simulink model "simulink_LenkmomentB"  (Simulink 6.5)
settings: Solver=ode5  StartTime=0.0  StopTime=15  FixedStep=0.001  RelTol=1e-3
PreLoadFcn:
  | global d
  | global p
undefined symbols (not defined in the file or in its folder): d, p, x
settings Model: Creator=tftbe1  LastModifiedBy=localadmin
settings OptimizationCC: InitFltsAndDblsToZero=off
settings DebuggingCC: SignalResolutionControl=UseLocalSettings  StrictBusMsg=ErrorLevel1
settings GRTTargetCC: TargetFcnLib=ansi_tfl_table_tmw.mat

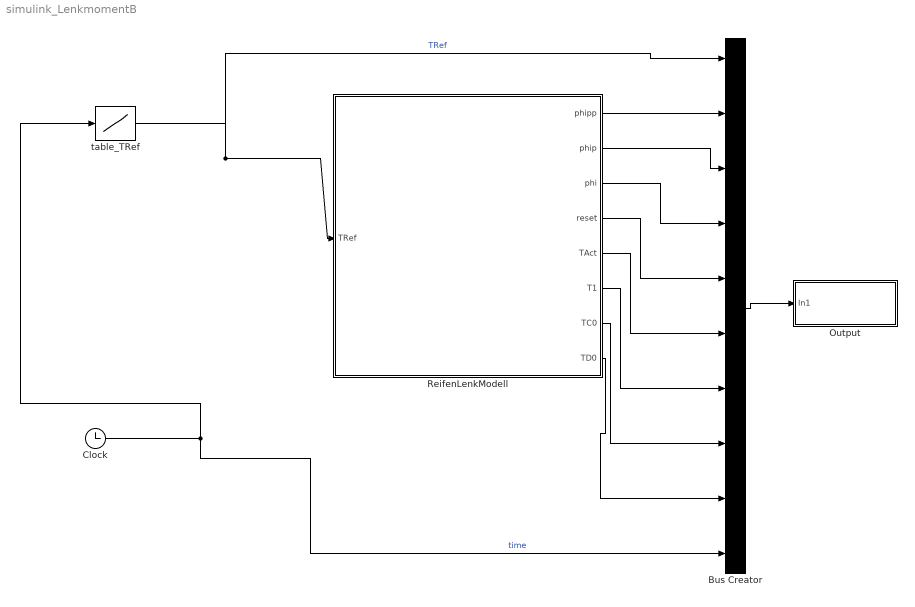
== system simulink_LenkmomentB ==
  Bus Creator : BusCreator  Inputs=10
  Clock : Clock
      settings: Decimation=10
  Output : Subsystem
  ReifenLenkModell : Subsystem
  table_TRef : Lookup  InputValues=d.time  OutputValues=d.IPAS_Soll_Lenkmoment  LookUpMeth=Interpolation-Extrapolation  OutDataType=sfix(16)  OutScaling=2^0  SampleTime=-1  LUTDesignTableMode=Redesign Table  LUTDesignDataSource=Block Dialog  LUTDesignFunctionName=sqrt(x)  LUTDesignUseExistingBP=on  LUTDesignRelError=0.01  LUTDesignAbsError=1e-6  SaturateOnIntegerOverflow=off  RndMeth=Floor
      settings: LockScale=off
  wires:
  Bus Creator/1 -> Output/1(In1)
  ReifenLenkModell/1(phipp) -> Bus Creator/2
  ReifenLenkModell/2(phip) -> Bus Creator/3
  ReifenLenkModell/3(phi) -> Bus Creator/4
  Clock/1 -> table_TRef/1, Bus Creator/10  "time"
  table_TRef/1 -> ReifenLenkModell/1(TRef), Bus Creator/1  "TRef"
  ReifenLenkModell/4(reset) -> Bus Creator/5
  ReifenLenkModell/5(TAct) -> Bus Creator/6
  ReifenLenkModell/6(T1) -> Bus Creator/7
  ReifenLenkModell/7(TC0) -> Bus Creator/8
  ReifenLenkModell/8(TD0) -> Bus Creator/9

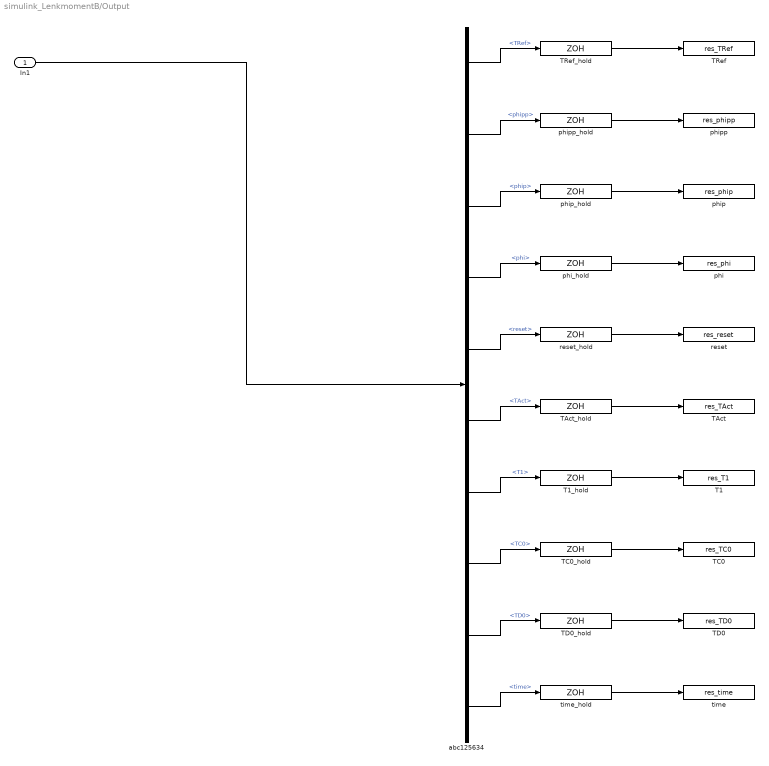
== system simulink_LenkmomentB/Output ==
  In1 : Inport
  T1 : ToWorkspace  VariableName=res_T1  SampleTime=-1  SaveFormat=Array
  T1_hold : ZeroOrderHold  SampleTime=0.01
  TAct : ToWorkspace  VariableName=res_TAct  SampleTime=-1  SaveFormat=Array
  TAct_hold : ZeroOrderHold  SampleTime=0.01
  TC0 : ToWorkspace  VariableName=res_TC0  SampleTime=-1  SaveFormat=Array
  TC0_hold : ZeroOrderHold  SampleTime=0.01
  TD0 : ToWorkspace  VariableName=res_TD0  SampleTime=-1  SaveFormat=Array
  TD0_hold : ZeroOrderHold  SampleTime=0.01
  TRef : ToWorkspace  VariableName=res_TRef  SampleTime=-1  SaveFormat=Array
  TRef_hold : ZeroOrderHold  SampleTime=0.01
  abc125634 : BusSelector  OutputSignals=TRef,phipp,phip,phi,reset,TAct,T1,TC0,TD0,time
  phi : ToWorkspace  VariableName=res_phi  SampleTime=-1  SaveFormat=Array
  phi_hold : ZeroOrderHold  SampleTime=0.01
  phip : ToWorkspace  VariableName=res_phip  SampleTime=-1  SaveFormat=Array
  phip_hold : ZeroOrderHold  SampleTime=0.01
  phipp : ToWorkspace  VariableName=res_phipp  SampleTime=-1  SaveFormat=Array
  phipp_hold : ZeroOrderHold  SampleTime=0.01
  reset : ToWorkspace  VariableName=res_reset  SampleTime=-1  SaveFormat=Array
  reset_hold : ZeroOrderHold  SampleTime=0.01
  time : ToWorkspace  VariableName=res_time  SampleTime=-1  SaveFormat=Array
  time_hold : ZeroOrderHold  SampleTime=0.01
  wires:
  In1/1 -> abc125634/1
  abc125634/1 -> TRef_hold/1  "<TRef>"
  TRef_hold/1 -> TRef/1
  abc125634/2 -> phipp_hold/1  "<phipp>"
  phipp_hold/1 -> phipp/1
  abc125634/3 -> phip_hold/1  "<phip>"
  phip_hold/1 -> phip/1
  abc125634/4 -> phi_hold/1  "<phi>"
  phi_hold/1 -> phi/1
  abc125634/5 -> reset_hold/1  "<reset>"
  reset_hold/1 -> reset/1
  abc125634/6 -> TAct_hold/1  "<TAct>"
  TAct_hold/1 -> TAct/1
  abc125634/7 -> T1_hold/1  "<T1>"
  T1_hold/1 -> T1/1
  abc125634/8 -> TC0_hold/1  "<TC0>"
  TC0_hold/1 -> TC0/1
  abc125634/9 -> TD0_hold/1  "<TD0>"
  TD0_hold/1 -> TD0/1
  abc125634/10 -> time_hold/1  "<time>"
  time_hold/1 -> time/1

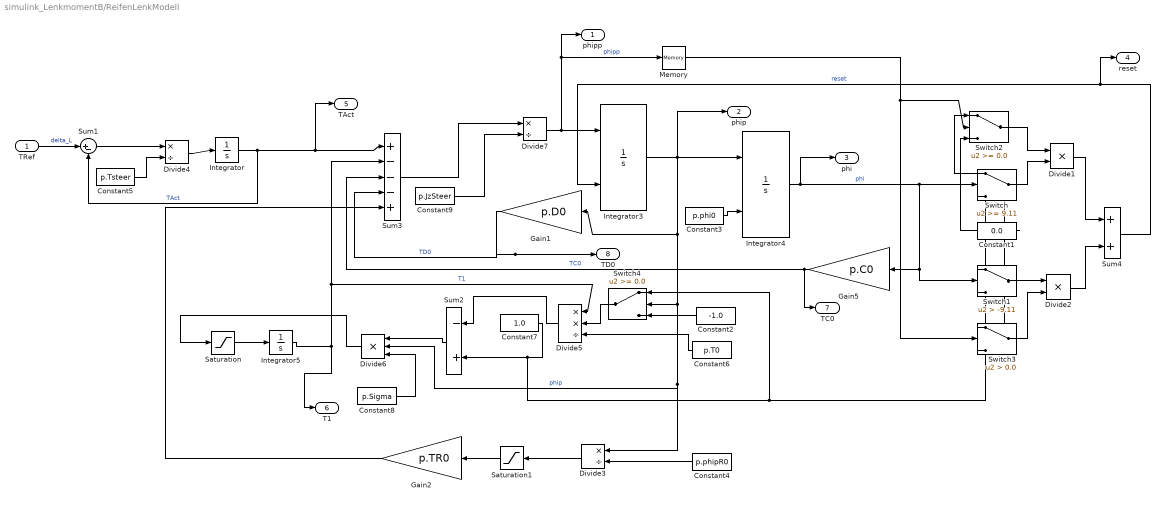
== system simulink_LenkmomentB/ReifenLenkModell ==
  TRef : Inport
  Constant1 : Constant  Value=0.0  OutDataType=sfix(16)  ConRadixGroup=Use specified scaling  OutScaling=2^0  SampleTime=inf  FramePeriod=inf
  Constant2 : Constant  Orientation=left  Value=-1.0  OutDataType=sfix(16)  ConRadixGroup=Use specified scaling  OutScaling=2^0  SampleTime=inf  FramePeriod=inf
  Constant3 : Constant  Value=p.phi0  OutDataType=sfix(16)  ConRadixGroup=Use specified scaling  OutScaling=2^0  SampleTime=inf  FramePeriod=inf
  Constant4 : Constant  Orientation=left  Value=p.phipR0  OutDataType=sfix(16)  ConRadixGroup=Use specified scaling  OutScaling=2^0  SampleTime=inf  FramePeriod=inf
  Constant5 : Constant  Value=p.Tsteer  OutDataType=sfix(16)  ConRadixGroup=Use specified scaling  OutScaling=2^0  SampleTime=inf  FramePeriod=inf
  Constant6 : Constant  Orientation=left  Value=p.T0  OutDataType=sfix(16)  ConRadixGroup=Use specified scaling  OutScaling=2^0  SampleTime=inf  FramePeriod=inf
  Constant7 : Constant  Value=1.0  OutDataType=sfix(16)  ConRadixGroup=Use specified scaling  OutScaling=2^0  SampleTime=inf  FramePeriod=inf
  Constant8 : Constant  Value=p.Sigma  OutDataType=sfix(16)  ConRadixGroup=Use specified scaling  OutScaling=2^0  SampleTime=inf  FramePeriod=inf
  Constant9 : Constant  Value=p.JzSteer  OutDataType=sfix(16)  ConRadixGroup=Use specified scaling  OutScaling=2^0  SampleTime=inf  FramePeriod=inf
  Divide1 : Product  Inputs=**
  Divide2 : Product  Inputs=**
  Divide3 : Product  Orientation=left  Inputs=*/
  Divide4 : Product  Inputs=*/
  Divide5 : Product  Orientation=left  Inputs=**/
  Divide6 : Product  Orientation=left  Inputs=***
  Divide7 : Product  Inputs=*/
  Gain1 : Gain  Orientation=left  Gain=p.D0
  Gain2 : Gain  Orientation=left  Gain=p.TR0
  Gain5 : Gain  Orientation=left  Gain=p.C0
  Integrator : Integrator  InitialCondition=0.0
  Integrator3 : Integrator  ExternalReset=level  InitialCondition=0.0
  Integrator4 : Integrator  InitialConditionSource=external  InitialCondition=0.0
  Integrator5 : Integrator  InitialCondition=0.0
  Memory : Memory
  Saturation : Saturate  UpperLimit=10000000  LowerLimit=-10000000
  Saturation1 : Saturate  Orientation=left  UpperLimit=1.0  LowerLimit=-1.0
  Sum1 : Sum  Inputs=|+-
  Sum2 : Sum  Orientation=left  Inputs=-+
  Sum3 : Sum  Inputs=+---+
  Sum4 : Sum
  Switch : Switch  Threshold=9.11
  Switch1 : Switch  Criteria=u2 > Threshold  Threshold=-9.11
  Switch2 : Switch  Threshold=0.0
  Switch3 : Switch  Criteria=u2 > Threshold  Threshold=0.0
  Switch4 : Switch  Orientation=left  Threshold=0.0
  phipp : Outport
  phip : Outport  Port=2
  phi : Outport  Port=3
  reset : Outport  Port=4
  TAct : Outport  Port=5
  T1 : Outport  Port=6
  TC0 : Outport  Port=7
  TD0 : Outport  Port=8
  wires:
  Integrator/1 -> Sum1/2, Sum3/1, TAct/1  "TAct"
  TRef/1 -> Sum1/1  "delta_L"
  Sum1/1 -> Divide4/1
  Constant5/1 -> Divide4/2
  Divide4/1 -> Integrator/1
  Integrator3/1 -> Integrator4/1, phip/1, Switch4/2, Divide6/2, Divide3/1, Gain1/1  "phip"
  Constant6/1 -> Divide5/3
  Switch4/1 -> Divide5/2
  Integrator5/1 -> Divide5/1, Sum3/2, T1/1  "T1"
  Constant7/1 -> Sum2/2, Switch1/3, Switch/1, Switch2/1, Switch3/3, Switch4/1
  Divide5/1 -> Sum2/1
  Sum2/1 -> Divide6/1
  Divide6/1 -> Saturation/1
  Constant8/1 -> Divide6/3
  Integrator4/1 -> Switch/2, Gain5/1, Switch1/2, phi/1  "phi"
  Gain5/1 -> Sum3/3, TC0/1  "TC0"
  Sum3/1 -> Divide7/1
  Constant9/1 -> Divide7/2
  Divide7/1 -> Integrator3/1, Memory/1, phipp/1  "phipp"
  Constant1/1 -> Switch/3, Switch2/3, Switch1/1, Switch3/1
  Sum4/1 -> Integrator3/2, reset/1  "reset"
  Switch2/1 -> Divide1/1
  Switch/1 -> Divide1/2
  Divide1/1 -> Sum4/1
  Memory/1 -> Switch2/2, Switch3/2
  Divide2/1 -> Sum4/2
  Switch1/1 -> Divide2/1
  Switch3/1 -> Divide2/2
  Gain1/1 -> Sum3/4, TD0/1  "TD0"
  Constant2/1 -> Switch4/3
  Constant3/1 -> Integrator4/2
  Saturation/1 -> Integrator5/1
  Constant4/1 -> Divide3/2
  Divide3/1 -> Saturation1/1
  Saturation1/1 -> Gain2/1
  Gain2/1 -> Sum3/5
